simulink model "clik_jacobian_pseudoinverse"  (R2024b)
settings: Solver=VariableStepAuto  StartTime=0.0  StopTime=24*5  RelTol=1e-3
undefined symbols (not defined in the file or in its folder): DiscIntNeverNeededParam, k0, K_pinv, q0, Tc
settings Model: Creator=Valentina Giannotti  LastModifiedBy=giaco
settings OptimizationCC: ReuseModelBlockBuffer=off
settings RTWCC: GPUComputeCapability=3.5

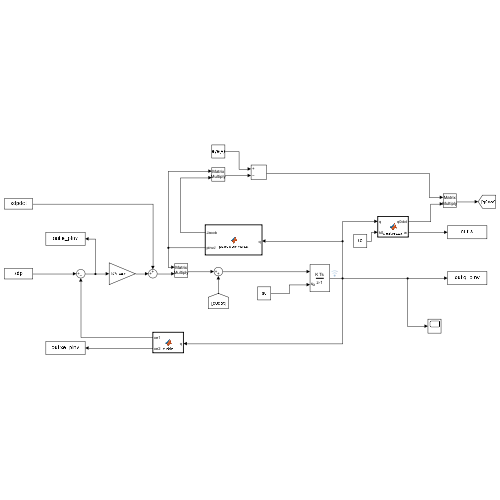
[thumbnail: Simulink's stored preview of the top-level diagram]
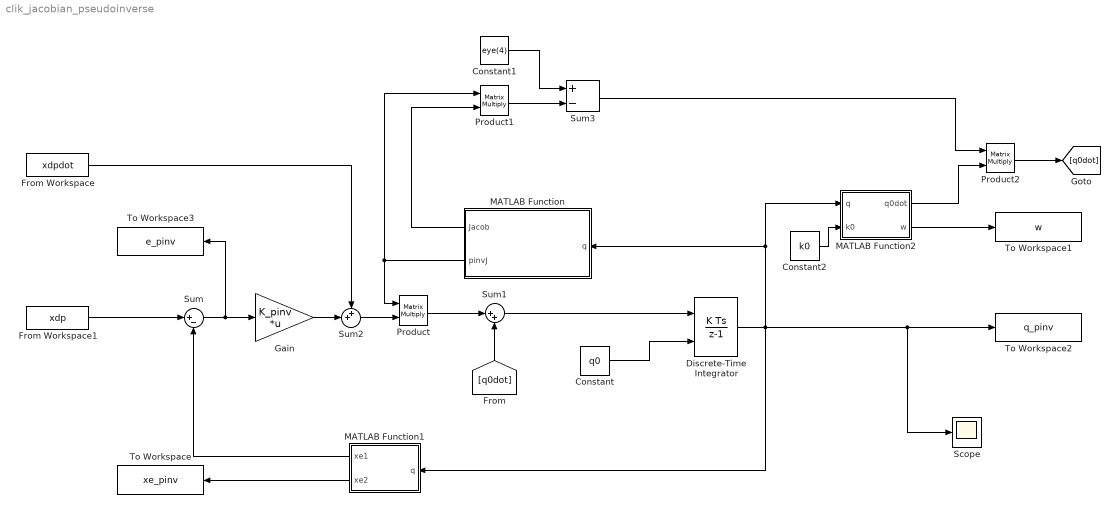
== system clik_jacobian_pseudoinverse ==
  Constant : Constant  Value=q0
  Constant1 : Constant  Value=eye(4)
  Constant2 : Constant  Value=k0
  Discrete-Time Integrator : DiscreteIntegrator  InitialConditionSource=external  InitialCondition=[0 -pi/2 -0.5 pi/2]'  SampleTime=Tc  ICPrevOutput=DiscIntNeverNeededParam  ICPrevScaledInput=DiscIntNeverNeededParam
  From Workspace : FromWorkspace  VariableName=xdpdot  SampleTime=Tc
  From Workspace1 : FromWorkspace  VariableName=xdp  SampleTime=Tc
  Gain : Gain  Gain=K_pinv  Multiplication=Matrix(K*u) (u vector)
  MATLAB Function : MATLAB Function  TreatAsAtomicUnit=on
  MATLAB Function1 : MATLAB Function  TreatAsAtomicUnit=on
  MATLAB Function2 : MATLAB Function  TreatAsAtomicUnit=on
  Product : Product  Multiplication=Matrix(*)
  Product1 : Product  Multiplication=Matrix(*)
  Product2 : Product  Multiplication=Matrix(*)
  Scope : Scope
  Sum : Sum  Inputs=|+-
  Sum1 : Sum  Inputs=|++
  Sum2 : Sum  Inputs=++|
  Sum3 : Sum  Inputs=+-
  To Workspace : ToWorkspace  VariableName=xe_pinv  SaveFormat=Structure With Time  SampleTime=-1
  To Workspace1 : ToWorkspace  VariableName=w  SaveFormat=Structure With Time  SampleTime=-1
  To Workspace2 : ToWorkspace  VariableName=q_pinv  SaveFormat=Structure With Time  SampleTime=-1
  To Workspace3 : ToWorkspace  VariableName=e_pinv  SaveFormat=Structure With Time  SampleTime=-1
  wires:
  Product1/1 -> Sum3/2
  MATLAB Function2/2(w) -> To Workspace1/1
  Constant2/1 -> MATLAB Function2/2(k0)
  From Workspace1/1 -> Sum/1
  Product2/1 -> [q0dot]
  MATLAB Function/1(Jacob) -> Product1/2
  MATLAB Function2/1(q0dot) -> Product2/2
  MATLAB Function/2(pinvJ) -> Product1/1, Product/1
  Constant1/1 -> Sum3/1
  Discrete-Time Integrator/1 -> MATLAB Function2/1(q), MATLAB Function/1(q), MATLAB Function1/1(q), Scope/1, To Workspace2/1
  [q0dot] -> Sum1/2
  Sum3/1 -> Product2/1
  Sum2/1 -> Product/2
  MATLAB Function1/2(xe2) -> To Workspace/1
  Constant/1 -> Discrete-Time Integrator/2
  Product/1 -> Sum1/1
  From Workspace/1 -> Sum2/1
  Sum1/1 -> Discrete-Time Integrator/1
  Sum/1 -> To Workspace3/1, Gain/1
  MATLAB Function1/1(xe1) -> Sum/2
  Gain/1 -> Sum2/2

== matlab function clik_jacobian_pseudoinverse/MATLAB Function ==
  data: Jacob output; pinvJ output; q input
function [Jacob,pinvJ]=pseudoinversa(q)
% Drop the z row so the task only constrains x, y, and yaw.
a1=0.5;
a2=a1;

Jacob=[-a1*sin(q(1))-a2*sin(q(1)+q(2)) -a2*sin(q(1)+q(2)),0,0;
      a1*cos(q(1))+a2*cos(q(1)+q(2))  a2*cos(q(1)+q(2)),0,0;
    1,1,0,1];

pinvJ=pinv(Jacob);
end

== matlab function clik_jacobian_pseudoinverse/MATLAB Function2 ==
  data: q input; q0dot output; k0 input; w output
function [q0dot ,w] = destrezza(q,k0)
% Use the gradient of sin(q2)^2 to steer away from planar singularities.

w=(sin(q(2)))^2;
dw=[0 2*sin(q(2))*cos(q(2)) 0 0]';

q0dot=k0*dw;

end

== matlab function clik_jacobian_pseudoinverse/MATLAB Function1 ==
  data: q input; xe1 output; xe2 output
function [xe1, xe2] = dirkin(q)
% Return the reduced task coordinates and the full pose for plotting.
a1=0.5;
a2=a1;
d0=1;

xe1=[a1*cos(q(1))+a2*cos(q(1)+q(2));...
    a1*sin(q(1))+a2*sin(q(1)+q(2));...
    q(1)+q(2)+q(4)];

xe2=[a1*cos(q(1))+a2*cos(q(1)+q(2));...
    a1*sin(q(1))+a2*sin(q(1)+q(2));...
    d0+q(3);...
    q(1)+q(2)+q(4)];
end
